simulink model "rsw_arm6"  (R2025b)
settings: Solver=VariableStepAuto  StartTime=0.0  StopTime=5  RelTol=1e-3
settings Model: Creator=31634  LastModifiedBy=31634

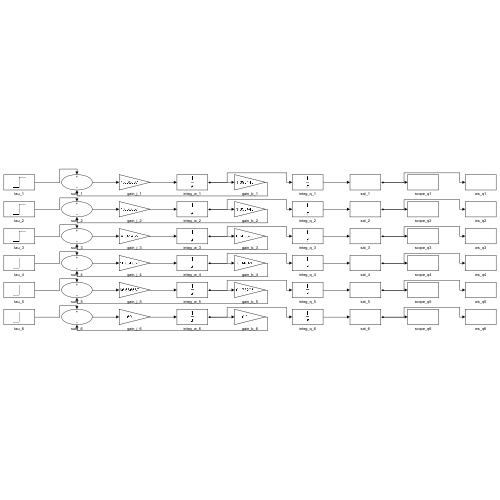
[thumbnail: Simulink's stored preview of the top-level diagram]
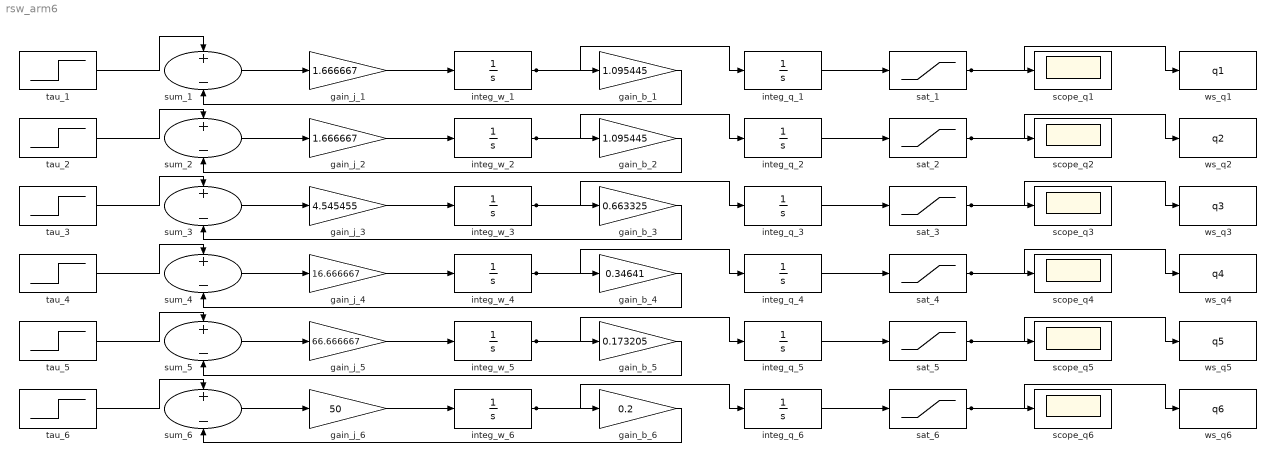
== system rsw_arm6 ==
  gain_b_1 : Gain  Gain=1.095445
  gain_b_2 : Gain  Gain=1.095445
  gain_b_3 : Gain  Gain=0.663325
  gain_b_4 : Gain  Gain=0.34641
  gain_b_5 : Gain  Gain=0.173205
  gain_b_6 : Gain  Gain=0.2
  gain_j_1 : Gain  Gain=1.666667
  gain_j_2 : Gain  Gain=1.666667
  gain_j_3 : Gain  Gain=4.545455
  gain_j_4 : Gain  Gain=16.666667
  gain_j_5 : Gain  Gain=66.666667
  gain_j_6 : Gain  Gain=50
  integ_q_{1..6} (6 alike) : Integrator
  integ_w_{1..6} (6 alike) : Integrator
  sat_1 : Saturate  UpperLimit=2.96706  LowerLimit=-2.96706
  sat_2 : Saturate  UpperLimit=1.919862  LowerLimit=-1.919862
  sat_3 : Saturate  UpperLimit=2.617994  LowerLimit=-2.617994
  sat_4 : Saturate  UpperLimit=3.141593  LowerLimit=-3.141593
  sat_5 : Saturate  UpperLimit=2.094395  LowerLimit=-2.094395
  sat_6 : Saturate  UpperLimit=3.141593  LowerLimit=-3.141593
  scope_q{1..6} (6 alike) : Scope
  sum_{1..6} (6 alike) : Sum  Inputs=+-
  tau_{1..6} (6 alike) : Step  Time=0.1  SampleTime=0
  ws_q1 : ToWorkspace  VariableName=q1  SampleTime=-1
  ws_q2 : ToWorkspace  VariableName=q2  SampleTime=-1
  ws_q3 : ToWorkspace  VariableName=q3  SampleTime=-1
  ws_q4 : ToWorkspace  VariableName=q4  SampleTime=-1
  ws_q5 : ToWorkspace  VariableName=q5  SampleTime=-1
  ws_q6 : ToWorkspace  VariableName=q6  SampleTime=-1
  wires:
  sat_1/1 -> ws_q1/1, scope_q1/1
  tau_1/1 -> sum_1/1
  integ_w_1/1 -> gain_b_1/1, integ_q_1/1
  gain_b_1/1 -> sum_1/2
  sum_1/1 -> gain_j_1/1
  gain_j_1/1 -> integ_w_1/1
  integ_q_1/1 -> sat_1/1
  sat_2/1 -> ws_q2/1, scope_q2/1
  tau_2/1 -> sum_2/1
  integ_w_2/1 -> gain_b_2/1, integ_q_2/1
  gain_b_2/1 -> sum_2/2
  sum_2/1 -> gain_j_2/1
  gain_j_2/1 -> integ_w_2/1
  integ_q_2/1 -> sat_2/1
  sat_3/1 -> ws_q3/1, scope_q3/1
  tau_3/1 -> sum_3/1
  integ_w_3/1 -> gain_b_3/1, integ_q_3/1
  gain_b_3/1 -> sum_3/2
  sum_3/1 -> gain_j_3/1
  gain_j_3/1 -> integ_w_3/1
  integ_q_3/1 -> sat_3/1
  sat_4/1 -> ws_q4/1, scope_q4/1
  tau_4/1 -> sum_4/1
  integ_w_4/1 -> gain_b_4/1, integ_q_4/1
  gain_b_4/1 -> sum_4/2
  sum_4/1 -> gain_j_4/1
  gain_j_4/1 -> integ_w_4/1
  integ_q_4/1 -> sat_4/1
  sat_5/1 -> ws_q5/1, scope_q5/1
  tau_5/1 -> sum_5/1
  integ_w_5/1 -> gain_b_5/1, integ_q_5/1
  gain_b_5/1 -> sum_5/2
  sum_5/1 -> gain_j_5/1
  gain_j_5/1 -> integ_w_5/1
  integ_q_5/1 -> sat_5/1
  sat_6/1 -> ws_q6/1, scope_q6/1
  tau_6/1 -> sum_6/1
  integ_w_6/1 -> gain_b_6/1, integ_q_6/1
  gain_b_6/1 -> sum_6/2
  sum_6/1 -> gain_j_6/1
  gain_j_6/1 -> integ_w_6/1
  integ_q_6/1 -> sat_6/1
